simulink model "uart"  (R2025a)
settings: Solver=FixedStepAuto  StartTime=0.0  StopTime=50  FixedStep=0.1  RelTol=1e-3
InitFcn:
  | run('param_init.m')
values from neighbouring files (symbols this model uses):
  Cd = [0.0357; 0.0763; 1.4515]    [param_init.m]
  Cl = [0.2; 4.8]    [param_init.m]
  g = 9.80665    [get_rho.m]    (also in param_init.m = 9.81)
  initTAS = 66.5    [param_init.m]
  M = 0.0289652    [get_rho.m]    (also in param_init.m = 2994)
  rho = p0*M/(R*T0)*(1 - L*h/T0).^(g*M/(R*L) - 1)    [get_rho.m]    (also in param_init.m = get_rho(altitude))
  S = 30.19    [param_init.m]
undefined symbols (not defined in the file or in its folder): NULL
libraries: instrumentseriallib x3, svdutilitieslib x1
settings Model: Creator=Martin  LastModifiedBy=LUONG KIEU
settings DebuggingCC: UnconnectedInputMsg=warning  UnconnectedOutputMsg=warning  UnconnectedLineMsg=warning
settings ModelReferenceCC: EnableRefExpFcnMdlSchedulingChecks=on
settings RTWCC: GPUComputeCapability=3.5  DLArmComputeVersion=19.05

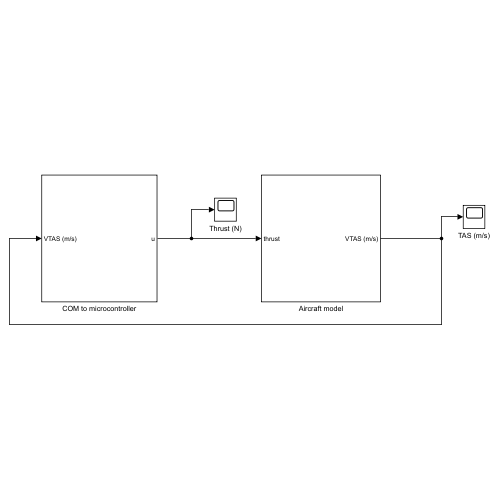
[thumbnail: Simulink's stored preview of the top-level diagram]
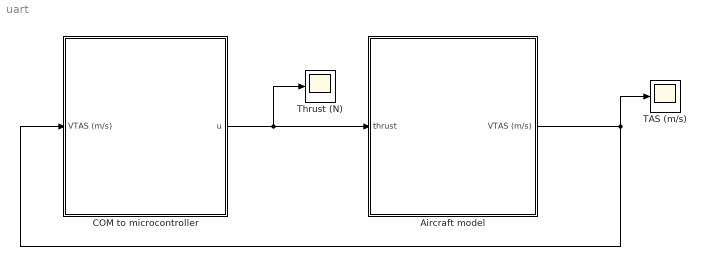
== system uart ==
  Aircraft model : Subsystem
  COM to microcontroller : Subsystem
  TAS (m/s) : Scope
      settings: ActiveDisplayYMinimum=64.55687  ActiveDisplayYMaximum=83.98819
  Thrust (N) : Scope
      settings: ActiveDisplayYMinimum=2233.87411  ActiveDisplayYMaximum=12639.44693
  wires:
  COM to microcontroller/1(u) -> Thrust (N)/1, Aircraft model/1(thrust)
  Aircraft model/1(VTAS (m/s)) -> COM to microcontroller/1(VTAS (m/s)), TAS (m/s)/1

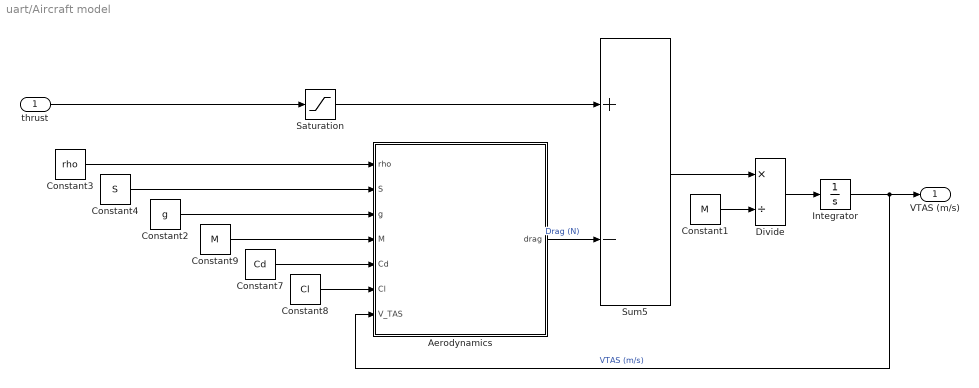
== system uart/Aircraft model ==
  thrust : Inport
  Aerodynamics : Subsystem
  Constant1 : Constant  Value=M
  Constant2 : Constant  Value=g
  Constant3 : Constant  Value=rho
  Constant4 : Constant  Value=S
  Constant7 : Constant  Value=Cd
  Constant8 : Constant  Value=Cl
  Constant9 : Constant  Value=M
  Divide : Product  Inputs=*/
  Integrator : Integrator  InitialCondition=initTAS  LimitOutput=on  UpperSaturationLimit=250  LowerSaturationLimit=30
  Saturation : Saturate  UpperLimit=10000  LowerLimit=0
  Sum5 : Sum  Inputs=+-
  VTAS (m/s) : Outport
  wires:
  Constant8/1 -> Aerodynamics/6(Cl)
  Constant7/1 -> Aerodynamics/5(Cd)
  Constant9/1 -> Aerodynamics/4(M)
  Constant4/1 -> Aerodynamics/2("S ")
  Saturation/1 -> Sum5/1
  Constant2/1 -> Aerodynamics/3(g)
  Constant3/1 -> Aerodynamics/1(rho)
  Sum5/1 -> Divide/1
  thrust/1 -> Saturation/1
  Constant1/1 -> Divide/2
  Aerodynamics/1(drag) -> Sum5/2  "Drag (N)"
  Integrator/1 -> Aerodynamics/7(V_TAS), VTAS (m/s)/1  "VTAS (m/s)"
  Divide/1 -> Integrator/1

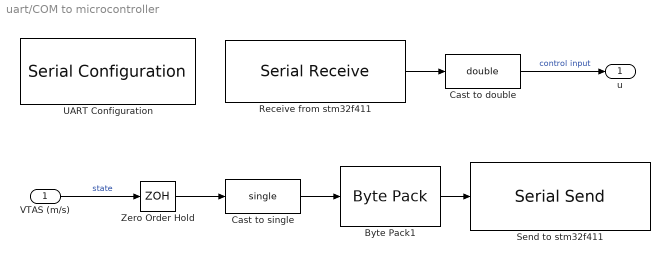
== system uart/COM to microcontroller ==
  VTAS (m/s) : Inport
  " Cast to double" : DataTypeConversion  OutDataTypeStr=double  SaturateOnIntegerOverflow=off  RndMeth=Floor
  Byte Pack1 : svdutilitieslib/Byte Pack  maskPackedDataType=uint32  datatypes={'single'}  byteAlign=4  blockPlatform=arduinoert
  Cast to single : DataTypeConversion  OutDataTypeStr=single  SaturateOnIntegerOverflow=off  RndMeth=Floor
  Receive from stm32f411 : instrumentseriallib/Serial Receive  Priority=2  PortSel=COM7  Port=COM7  ComPort=COM7  DataType=single  SaveDataType=uint8  ToggleHeader=on  Header='H'  ToggleDataSize=on  DataSize=[1 1]  ToggleTerminator=on  Terminator=NULL ('\0')  CustomTerminator=[]  InputFormat=Column major  EnableBlockingMode=on  ActionDataUnavailable=Output last received value  ActionWhenDataUnavailable=Output last received value  CustomValue=0  SampleTime=0.1  SimulateUsing=Interpreted execution  BlockInModel=on  aMode=1  LibraryInUse=instrumentlib
  Send to stm32f411 : instrumentseriallib/Serial Send  Priority=1  PortSel=COM7  Port=COM7  ComPort=COM7  Header=[]  Terminator=<none>  CustomTerminator=[]  EnableBlockingMode=on  SimulateUsing=Interpreted execution  BlockInModel=on  aMode=1
  UART Configuration : instrumentseriallib/Serial Configuration  Priority=-200000  PortSel=COM7  Port=COM7  ComPort=COM7  BaudRate=38400  DataBits=8  Parity=none  StopBits=1  ByteOrder=little-endian  FlowControl=none  Timeout=10  SimulateUsing=Interpreted execution  BlockInModel=on  aMode=1
  Zero Order Hold : ZeroOrderHold  SampleTime=0.1
  u : Outport
  wires:
  " Cast to double"/1 -> u/1  "control input"
  VTAS (m/s)/1 -> Zero Order Hold/1  "state"
  Zero Order Hold/1 -> Cast to single/1
  Cast to single/1 -> Byte Pack1/1
  Byte Pack1/1 -> Send to stm32f411/1
  Receive from stm32f411/1 -> " Cast to double"/1

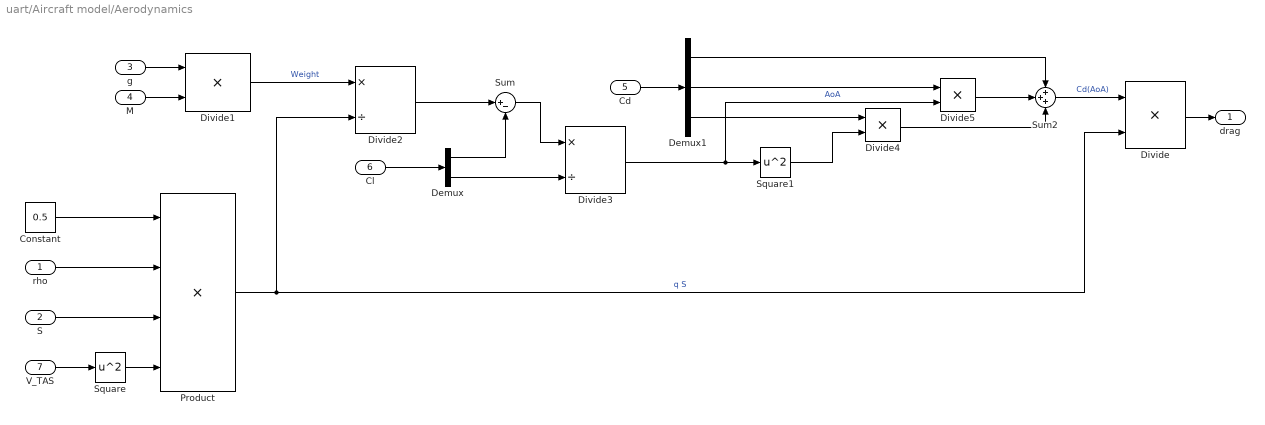
== system uart/Aircraft model/Aerodynamics ==
  rho : Inport
  "S " : Inport  Port=2
  g : Inport  Port=3
  M : Inport  Port=4
  Cd : Inport  Port=5
  Cl : Inport  Port=6
  V_TAS : Inport  Port=7
  Constant : Constant  Value=0.5
  Demux : Demux  Outputs=2
  Demux1 : Demux  Outputs=3
  Divide{,1,4..5} (4 alike) : Product  Inputs=**
  Divide2 : Product  Inputs=*/
  Divide3 : Product  Inputs=*/
  Product : Product  Inputs=4
  Square : Math  Operator=square
  Square1 : Math  Operator=square
  Sum : Sum  Inputs=|+-
  Sum2 : Sum  Inputs=+++
  drag : Outport
  wires:
  Product/1 -> Divide/2, Divide2/2  "q S"
  Constant/1 -> Product/1
  rho/1 -> Product/2
  "S "/1 -> Product/3
  V_TAS/1 -> Square/1
  Square/1 -> Product/4
  g/1 -> Divide1/1
  M/1 -> Divide1/2
  Divide1/1 -> Divide2/1  "Weight"
  Divide2/1 -> Sum/1
  Cl/1 -> Demux/1
  Demux/1 -> Sum/2
  Sum/1 -> Divide3/1
  Demux/2 -> Divide3/2
  Divide3/1 -> Divide5/2, Square1/1  "AoA"
  Cd/1 -> Demux1/1
  Demux1/2 -> Divide5/1
  Demux1/1 -> Sum2/1
  Square1/1 -> Divide4/2
  Demux1/3 -> Divide4/1
  Divide5/1 -> Sum2/2
  Divide4/1 -> Sum2/3
  Sum2/1 -> Divide/1  "Cd(AoA)"
  Divide/1 -> drag/1
